simulink model "HFIAxisTest"  (R2026b)
settings: Solver=ode4  StopTime=hfiTestCfg.Duration  FixedStep=hfiTestCfg.PlantStep
PostLoadFcn:
  | addpath(fullfile(fileparts(get_param(bdroot,'FileName')),'..','build_process'));initialize_hfi_test(bdroot);
model workspace (MAT data in the model file):
  hfPlantCfg.Rs = 0.5
  hfPlantCfg.Ld = 0.001
  hfPlantCfg.Lq = 0.0015
  hfPlantCfg.Flux = 0.035
  hfPlantCfg.PolePairs = 4
  hfPlantCfg.J = 0.0005
  hfPlantCfg.B = 0.0001
  hfPlantCfg.Id0 = 0
  hfPlantCfg.Iq0 = 0
  hfPlantCfg.Speed0 = 0
  hfPlantCfg.Position0 = 0.175
  hfPlantCfg.SaturationDepth = 0
  hfPlantCfg.SaturationCurrent = 1
  hfPlantCfg.CrossInductance = 0
  hfPlantCfg.MechanicalEnabled = 1
  hfPlantCfg.Settings = [0.5; 0.001; 0.0015; 0.035; 4; 0.0005; 0.0001; 0; 1; 0; 1]
  hfPlantCfg.InitialState = [0; 0; 0; 0.175]
  hfiCfg.Ts = 5e-05
  hfiCfg.InjectionVoltage = 5
  hfiCfg.Ld = 0.001
  hfiCfg.Lq = 0.0015
  hfiCfg.CrossInductance = 0
  hfiCfg.InitialAxis = 0
  hfiCfg.MaxOmega = 80
  hfiCfg.MinVoltageStep = 1
  hfiCfg.MaxCrossFraction = 0.2
  hfiCfg.MinResponse = 0.01
  hfiCfg.MaxResponse = 0.15
  hfiCfg.MinInjectionScale = 0.1
  hfiCfg.DemodBandwidth = 300
  hfiCfg.DemodFilterEnabled = 1
  hfiCfg.UseMeasuredInverseAverage = 0
  hfiCfg.DemodA = 0.910057240676
  hfiCfg.InverseAverage = 833.333333333
  hfiCfg.CrossPhase = 0
  hfiCfg.InitialTrackerPhase = 0
  hfiCfg.AxisInitialState = [0; 0]
  hfiCfg.DemodSettings = [5e-05; 5; 833.333333333; 0; 1; 0.2; 0.01; 0.15; 0.1; 0.910057240676; 0]
  hfiCfg.TrackSettings = [0; 0; 80]
  hfiTestCfg.Duration = 0.25
  hfiTestCfg.Ts = 5e-05
  hfiTestCfg.PlantStep = 2.5e-06
  hfiTestCfg.InitialElectricalAngle = 0.7
  hfiTestCfg.InjectionScale = 1
  hfiTestCfg.Enable = 1
  hfiTestCfg.Reset = 0
  hfiTestCfg.LoadTorque = 0
  hfiTestCfg.MeasurementNoise = 0
  hfiTestCfg.NoiseSeed = 42
  hfiTestCfg.CurrentOffset = [0; 0; 0]
  hfiTestCfg.CurrentResolution = 0
  hfiTestCfg.CurrentRange = 8
  hfiTestCfg.CurrentDelay = 0
  hfiTestCfg.VoltageAlignmentDelay = 0
  hfiTestCfg.ExecutionDelay = 0
  hfiTestCfg.ActuationGain = 1
  hfiTestCfg.SaturationDepth = 0
  hfiTestCfg.CrossInductance = 0
  hfiTestCfg.MechanicalEnabled = 1
  hfiTestCfg.ExternalInverseAverage = 0
  pllCfg.Ts = 5e-05
  pllCfg.NaturalFrequency = 30
  pllCfg.Damping = 0.707
  pllCfg.Kp = 266.532720731
  pllCfg.Ki = 35530.5758439
  pllCfg.Kaw = 376.991118431
  pllCfg.OmegaMax = 160
  pllCfg.MinMagnitude = 0.01
  pllCfg.LockError = 0.12
  pllCfg.LockSamples = 100
  pllCfg.Theta0 = 0
  pllCfg.Omega0 = 0
  testStim.time = [0 5e-05 0.0001 0.00015 0.0002 0.00025 0.0003 0.00035 0.0004 0.00045 0.0005 0.00055 ... (5001 elements, 5001x1)]
  testStim.signals.values = [0 0 0 0 0 0 0 0 0 0 0 0 ... (35007 elements, 5001x7)]
  testStim.signals.dimensions = 7
libraries: ClarkePark x2, HighFrequencyObserver x1, PMSMHighFrequencyPlant x1
settings Model: Creator=24322  LastModifiedBy=24322

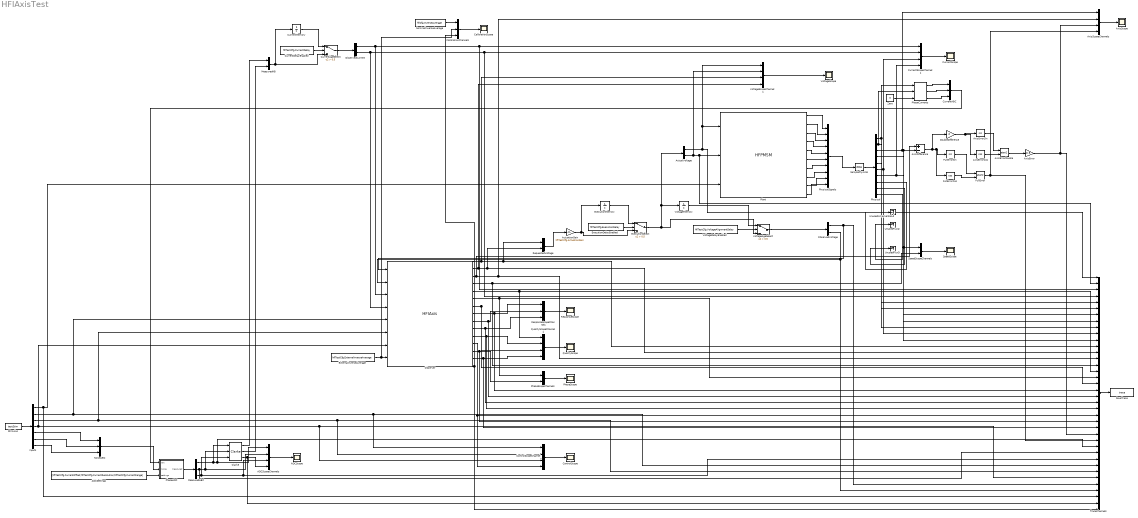
== system HFIAxisTest ==
  ADCScope : Scope
  ADCScopeChannels : Mux
  ADCSettings : Constant  Value=[hfiTestCfg.CurrentOffset;hfiTestCfg.CurrentResolution;hfiTestCfg.CurrentRange]
  ActualVoltage : Demux  Outputs=2
  ActuationGain : Gain  Gain=hfiTestCfg.ActuationGain
  AxisDifference : Sum  Inputs=+-
  AxisError : Gain  Gain=0.5
  AxisErrorCos : Trigonometry  Operator=cos
  AxisErrorDouble : Trigonometry  Operator=atan2
  AxisErrorSin : Trigonometry
  AxisScope : Scope
  AxisScopeChannels : Mux
  CalibrationChannels : Mux  Inputs=3
  CalibrationScope : Scope
  Clarke : ClarkePark/Clarke  SystemSampleTime=-1  VariantActivationTime=update diagram  EmptyChoice=off  PassThrough=off  PassThroughVariantControl=(default)  EmptyChoiceVariantControl=(default)  AllowFlexibleInterface=on  Latency=0  AutoFrameSizeCalculation=off
  ControlScope : Scope
  ControlScopeChannels : Mux
  CurrentABC : Mux  Inputs=3
  CurrentAgeSelect : Switch  Criteria=u2 > Threshold  Threshold=0.5  SaturateOnIntegerOverflow=off  InputSameDT=off
  CurrentDelayEnabled : Constant  Value=hfiTestCfg.CurrentDelay
  CurrentMemory : UnitDelay  InitialCondition=zeros(2,1)  SampleTime=hfiCfg.Ts
  CurrentScope : Scope
  CurrentScopeChannels : Mux
  DoubleDifference : Gain  Gain=2
  ExecutionDelayEnabled : Constant  Value=hfiTestCfg.ExecutionDelay
  ExecutionMemory : UnitDelay  InitialCondition=zeros(2,1)  SampleTime=hfiCfg.Ts
  ExecutionSelect : Switch  Criteria=u2 > Threshold  Threshold=0.5  SaturateOnIntegerOverflow=off  InputSameDT=off
  ExternalInverseAverage : Constant  Value=hfiTestCfg.ExternalInverseAverage
  FullError : Trigonometry  Operator=atan2
  FullErrorCos : Trigonometry  Operator=cos
  FullErrorSin : Trigonometry
  Inputs : Demux  Outputs=7
  MeasuredAB : Mux  Inputs=2
  MeasuredABC : Demux  Outputs=3
  NoiseABC : Mux  Inputs=3
  NominalInverseAverage : Constant  Value=hfiCfg.InverseAverage
  ObservedCurrent : Demux  Outputs=2
  ObservedVoltage : Demux  Outputs=2
  Observer : HighFrequencyObserver/HFIAxis  cfg=hfiCfg  trackerCfg=pllCfg
  PhaseADC : MATLAB Function  TreatAsAtomicUnit=on
  PhaseCurrents : ClarkePark/InverseClarke  SystemSampleTime=-1  VariantActivationTime=update diagram  EmptyChoice=off  PassThrough=off  PassThroughVariantControl=(default)  EmptyChoiceVariantControl=(default)  AllowFlexibleInterface=on  Latency=0  AutoFrameSizeCalculation=off
  PhaseScope : Scope
  PhaseScopeChannels : Mux  Inputs=2
  Physical : Demux  Outputs=10
  PhysicalSignals : Mux  Inputs=10
  Plant : PMSMHighFrequencyPlant/HFPMSM  cfg=hfPlantCfg
  QualityScope : Scope
  QualityScopeChannels : Mux
  RequestedVoltage : Mux  Inputs=2
  ResponseScope : Scope
  ResponseScopeChannels : Mux  Inputs=3
  SamplePhysical : ZeroOrderHold  SampleTime=hfiCfg.Ts
  SaveTrace : ToWorkspace  VariableName=trace  SaveFormat=Structure With Time  SampleTime=-1
  SpeedScope : Scope
  SpeedScopeChannels : Mux  Inputs=2
  Stimulus : FromWorkspace  VariableName=testStim  SampleTime=hfiCfg.Ts  Interpolate=off  OutputAfterFinalValue=Holding final value
  TraceChannels : Mux  Inputs=38
  UnusedFluxD : Terminator
  UnusedFluxQ : Terminator
  UnusedIncrementalLd : Terminator
  VoltageAgeSelect : Switch  Criteria=u2 > Threshold  Threshold=0.5  SaturateOnIntegerOverflow=off  InputSameDT=off
  VoltageDelayEnabled : Constant  Value=hfiTestCfg.VoltageAlignmentDelay
  VoltageMemory : UnitDelay  InitialCondition=zeros(2,1)  SampleTime=hfiCfg.Ts
  VoltageScope : Scope
  VoltageScopeChannels : Mux
  Zero : Constant  Value=0
  wires:
  Stimulus/1 -> Inputs/1
  ActuationGain/1 -> ExecutionMemory/1, ExecutionSelect/3
  ExecutionMemory/1 -> ExecutionSelect/1
  ExecutionDelayEnabled/1 -> ExecutionSelect/2
  RequestedVoltage/1 -> ActuationGain/1
  ExecutionSelect/1 -> ActualVoltage/1, VoltageMemory/1, VoltageAgeSelect/3
  VoltageMemory/1 -> VoltageAgeSelect/1
  VoltageDelayEnabled/1 -> VoltageAgeSelect/2
  VoltageAgeSelect/1 -> ObservedVoltage/1
  PhysicalSignals/1 -> SamplePhysical/1
  SamplePhysical/1 -> Physical/1
  CurrentABC/1 -> PhaseADC/1(raw)
  NoiseABC/1 -> PhaseADC/2(noise)
  ADCSettings/1 -> PhaseADC/3(settings)
  PhaseADC/1(measured) -> MeasuredABC/1
  MeasuredAB/1 -> CurrentAgeSelect/3, CurrentMemory/1
  CurrentMemory/1 -> CurrentAgeSelect/1
  CurrentDelayEnabled/1 -> CurrentAgeSelect/2
  CurrentAgeSelect/1 -> ObservedCurrent/1
  Zero/1 -> PhaseCurrents/3
  AxisDifference/1 -> FullErrorSin/1, FullErrorCos/1, DoubleDifference/1
  DoubleDifference/1 -> AxisErrorCos/1, AxisErrorSin/1
  AxisErrorSin/1 -> AxisErrorDouble/1
  AxisErrorCos/1 -> AxisErrorDouble/2
  AxisErrorDouble/1 -> AxisError/1
  FullErrorSin/1 -> FullError/1
  FullErrorCos/1 -> FullError/2
  TraceChannels/1 -> SaveTrace/1
  Inputs/1 -> TraceChannels/36, Plant/3
  Physical/1 -> PhaseCurrents/1, TraceChannels/5
  Physical/2 -> PhaseCurrents/2, TraceChannels/6
  Physical/3 -> TraceChannels/7, AxisDifference/2, AxisScopeChannels/1
  ActualVoltage/1 -> Plant/1, VoltageScopeChannels/1, TraceChannels/1
  Clarke/1 -> MeasuredAB/1
  ActualVoltage/2 -> TraceChannels/2, Plant/2, VoltageScopeChannels/2
  Clarke/2 -> MeasuredAB/2
  PhaseCurrents/1 -> CurrentABC/1
  MeasuredABC/1 -> TraceChannels/28, ADCScopeChannels/1, Clarke/1
  Inputs/5 -> NoiseABC/1
  PhaseCurrents/2 -> CurrentABC/2
  MeasuredABC/2 -> Clarke/2, ADCScopeChannels/2, TraceChannels/29
  Inputs/6 -> NoiseABC/2
  PhaseCurrents/3 -> CurrentABC/3
  MeasuredABC/3 -> TraceChannels/30, ADCScopeChannels/3, Clarke/3
  Inputs/7 -> NoiseABC/3
  Plant/1 -> PhysicalSignals/1
  Plant/2 -> PhysicalSignals/2
  Plant/3 -> PhysicalSignals/3
  Plant/4 -> PhysicalSignals/4
  Plant/5 -> PhysicalSignals/5
  Plant/6 -> PhysicalSignals/6
  Plant/7 -> PhysicalSignals/7
  Plant/8 -> PhysicalSignals/8
  Plant/9 -> PhysicalSignals/9
  Plant/10 -> PhysicalSignals/10
  Physical/4 -> TraceChannels/8, SpeedScopeChannels/1
  Physical/5 -> TraceChannels/9
  Physical/6 -> TraceChannels/10, CurrentScopeChannels/3
  Physical/7 -> TraceChannels/11, CurrentScopeChannels/4
  AxisError/1 -> AxisScopeChannels/3, TraceChannels/26
  FullError/1 -> AxisScopeChannels/4, TraceChannels/27
  Clarke/3 -> TraceChannels/37, ADCScopeChannels/4
  AxisScopeChannels/1 -> AxisScope/1
  SpeedScopeChannels/1 -> SpeedScope/1
  QualityScopeChannels/1 -> QualityScope/1
  VoltageScopeChannels/1 -> VoltageScope/1
  CurrentScopeChannels/1 -> CurrentScope/1
  ResponseScopeChannels/1 -> ResponseScope/1
  PhaseScopeChannels/1 -> PhaseScope/1
  ADCScopeChannels/1 -> ADCScope/1
  ControlScopeChannels/1 -> ControlScope/1
  Physical/10 -> UnusedFluxQ/1
  Physical/9 -> UnusedFluxD/1
  Physical/8 -> UnusedIncrementalLd/1
  CalibrationChannels/1 -> CalibrationScope/1
  NominalInverseAverage/1 -> CalibrationChannels/1
  Observer/15 -> CalibrationChannels/3, TraceChannels/38
  ExternalInverseAverage/1 -> CalibrationChannels/2, Observer/8
  Observer/14 -> QualityScopeChannels/4, TraceChannels/25
  Observer/13 -> PhaseScopeChannels/2, TraceChannels/24
  Observer/12 -> ControlScopeChannels/4, TraceChannels/23
  Observer/11 -> TraceChannels/22, QualityScopeChannels/2
  Observer/10 -> ResponseScopeChannels/3, TraceChannels/21
  Observer/9 -> TraceChannels/20, ResponseScopeChannels/2
  Observer/8 -> TraceChannels/19, ResponseScopeChannels/1
  Observer/7 -> TraceChannels/18, QualityScopeChannels/3
  Observer/6 -> TraceChannels/17, PhaseScopeChannels/1
  Observer/5 -> TraceChannels/16, QualityScopeChannels/1
  Observer/4 -> TraceChannels/15, SpeedScopeChannels/2
  ObservedCurrent/2 -> CurrentScopeChannels/2, TraceChannels/4, Observer/4
  ObservedVoltage/2 -> TraceChannels/35, Observer/2
  Observer/2 -> TraceChannels/13, RequestedVoltage/2, VoltageScopeChannels/4
  ObservedCurrent/1 -> CurrentScopeChannels/1, TraceChannels/3, Observer/3
  ObservedVoltage/1 -> TraceChannels/34, Observer/1
  Observer/1 -> TraceChannels/12, RequestedVoltage/1, VoltageScopeChannels/3
  Observer/3 -> AxisScopeChannels/2, TraceChannels/14, AxisDifference/1
  Inputs/4 -> ControlScopeChannels/3, TraceChannels/33, Observer/7
  Inputs/3 -> ControlScopeChannels/2, TraceChannels/32, Observer/6
  Inputs/2 -> ControlScopeChannels/1, TraceChannels/31, Observer/5

== matlab function HFIAxisTest/PhaseADC ==
  data: raw input; measured output; noise input; settings input
function measured=hfi_measure_current(raw,noise,settings)
%HFI_MEASURE_CURRENT Three phase ADC fixture: offset, noise, clipping, rounding.
% settings=[offset_a;offset_b;offset_c;resolution_A;range_A].
%#codegen
measured=min(max(raw+noise+settings(1:3),-settings(5)),settings(5));
if settings(4)>0
    measured=round(measured/settings(4))*settings(4);
end
end
